simulink model "dspic_model"  (Simulink 6.4)
settings: Solver=FixedStepDiscrete  StartTime=0.0  StopTime=10.0  FixedStep=0.001  RelTol=1e-3
libraries: dsPICdrivers x8, simulink x2
CloseFcn:
  | rtwprivate ssgencode ModelCloseRequest dspic_model
settings Model: LastModifiedBy=Philipp  BufferReuse=off  ProdHWDeviceType=16-bit Generic
settings OptimizationCC: BlockReduction=off  OptimizeBlockIOStorage=off  BufferReuse=off  EnforceIntegerDowncast=off  ExpressionFolding=off  LocalBlockOutputs=off  OptimizeModelRefInitCode=on  LifeSpan=1
settings HardwareCC: ProdBitPerInt=16  ProdEndianess=LittleEndian  ProdWordSize=16  ProdHWDeviceType=16-bit Generic  TargetHWDeviceType=32-bit Generic
settings RTWCC: SystemTargetFile=dspic.tlc  TemplateMakefile=dspic_pic30_gcc.tmf  PostCodeGenCommand=dsPIC_Compile()  Description=Embedded Target for Microchip dsPIC (real-time)  ProcessScript=dspic_make_rtw_hook
settings CodeAppCC: IgnoreCustomStorageClasses=off
settings STFCustomTargetCC: TargetFcnLib=ansi_tfl_tmw.mat  GenFloatMathFcnCalls=ANSI_C  ModelReferenceCompliant=off  IncludeMdlTerminateFcn=off  CombineOutputUpdateFcns=on  SuppressErrorStatus=on  IncludeERTFirstTime=on  ERTCustomFileBanners=on  SupportContinuousTime=off  SupportNonInlinedSFcns=off  SystemTargetFile=dspic.tlc
settings ERTTargetCC: TargetFcnLib=ansi_tfl_tmw.mat  GenFloatMathFcnCalls=ANSI_C  ModelReferenceCompliant=off  IncludeMdlTerminateFcn=off  SuppressErrorStatus=on  IncludeERTFirstTime=on  ERTFirstTimeCompliant=off  InlinedParameterPlacement=NonHierarchical  ERTSrcFileBannerTemplate=dsPIC_code_template.cgt  ERTHdrFileBannerTemplate=dsPIC_code_template.cgt  ERTDataSrcFileTemplate=dsPIC_code_template.cgt  ERTDataHdrFileTemplate=dsPIC_code_template.cgt  ERTCustomFileTemplate=dsPIC_main.tlc  InitialValueSource=Model
settings CustomProperty: DataType=string  Value=C:\PROGRA~1\MATLAB\R2006a\rtw\bin\win32\gmake

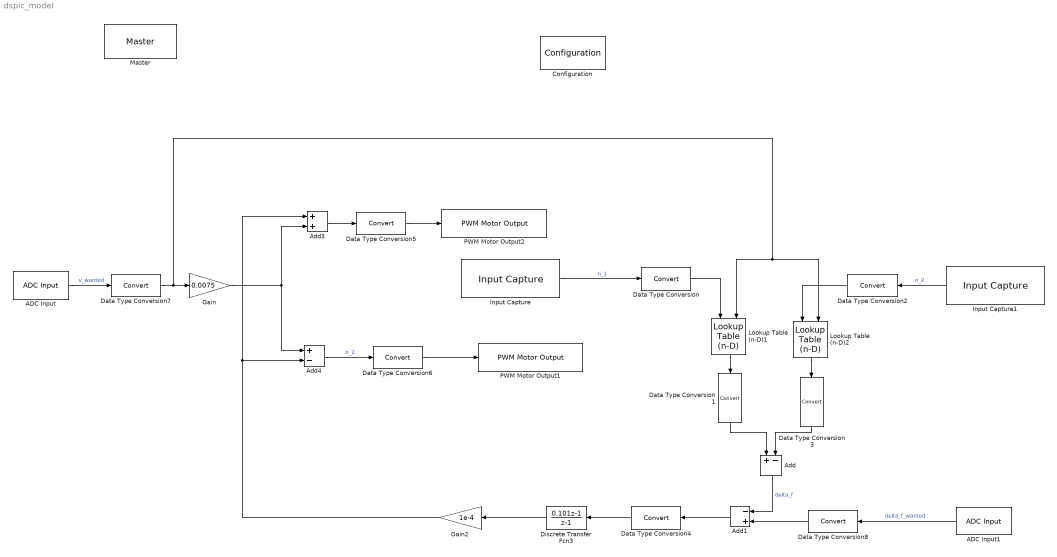
== system dspic_model ==
  ADC Input : dsPICdrivers/Peripheral I//O/ADC Input  Tag=dsPIC_ADC  Priority=5  ADC_TYPE=10 bits  ADC_MODE=Continuous sampling & get last channel value  NbrSampleStep=1  VoltRefpopup="AVdd  -  AVss"  OutFormatBitspopup=0000 00dd dddd dddd : Integer  InterruptPriority=6  ANCHANNELS=[0]  MaxName=ANmax = 1024  Rin=1e2  ADCS=0  SAMC=1  Temperature=25  SampleTime=0.001  Status="OK  |  Tsmp=5.000e-007 |  T/Channel=6.500e-006 |  Tall=6.500e-006"
  ADC Input1 : dsPICdrivers/Peripheral I//O/ADC Input  Tag=dsPIC_ADC  Orientation=left  Priority=5  ADC_TYPE=10 bits  ADC_MODE=Continuous sampling & get last channel value  NbrSampleStep=1  VoltRefpopup="AVdd  -  AVss"  OutFormatBitspopup=0000 00dd dddd dddd : Integer  InterruptPriority=6  ANCHANNELS=[1]  MaxName=ANmax = 1024  Rin=1e2  ADCS=0  SAMC=1  Temperature=25  SampleTime=0.001  Status="OK  |  Tsmp=5.000e-007 |  T/Channel=6.500e-006 |  Tall=6.500e-006"
  Add : Sum  Orientation=down  Inputs=+-  OutScaling=2^-10  SampleTime=0.001
  Add1 : Sum  Orientation=left  Inputs=-+  OutScaling=2^-10  SampleTime=0.001
  Add3 : Sum  OutScaling=2^-10  SampleTime=0.001
  Add4 : Sum  Inputs=+-  OutScaling=2^-10  SampleTime=0.001
  Configuration : dsPICdrivers/Configuration  SystemSampleTime=-1  double64=off
  Data Type Conversion : DataTypeConversion  OutDataTypeMode=double
  Data Type Conversion1 : DataTypeConversion  Orientation=down  OutDataTypeMode=uint16
  Data Type Conversion2 : DataTypeConversion  Orientation=left  OutDataTypeMode=double
  Data Type Conversion3 : DataTypeConversion  Orientation=down  OutDataTypeMode=uint16
  Data Type Conversion4 : DataTypeConversion  Orientation=left  OutDataTypeMode=double  SampleTime=0.001
  Data Type Conversion5 : DataTypeConversion  OutDataTypeMode=uint16  SampleTime=0.001
  Data Type Conversion6 : DataTypeConversion  OutDataTypeMode=uint16  SampleTime=0.001
  Data Type Conversion7 : DataTypeConversion  OutDataTypeMode=double  SampleTime=0.001
  Data Type Conversion8 : DataTypeConversion  Orientation=left  OutDataTypeMode=uint16  SampleTime=0.001
  Discrete Transfer Fcn3 : DiscreteTransferFcn  Orientation=left  Numerator=[0.101 -1]  Denominator=[1 -1]  SampleTime=0.001
  Gain : Gain  Gain=0.0075  SampleTime=0.001
  Gain2 : Gain  Orientation=left  Gain=1e-4  SampleTime=0.001
  Input Capture : dsPICdrivers/Peripheral I//O/Input Capture  Tag=dsPIC_PWM_IC  Priority=5  IntPriority=7  Channel=[ 1 ]  Channel_UP_Down_Periode=[4]  MaxChannel=[0.05]  SafeMarge=[10]  MaxName=' IC1max '  Precision=[15.6096]  Timer=[2]  ChangeDetected=[0]  ChangeDetectedPortRef=3  SampleTime=0.001  Status=OK
  Input Capture1 : dsPICdrivers/Peripheral I//O/Input Capture  Tag=dsPIC_PWM_IC  Orientation=left  Priority=5  IntPriority=7  Channel=[ 2 ]  Channel_UP_Down_Periode=[4]  MaxChannel=[0.05]  SafeMarge=[10]  MaxName=' IC2max '  Precision=[15.6096]  Timer=[2]  ChangeDetected=[0]  ChangeDetectedPortRef=3  SampleTime=0.001  Status=OK
  Lookup Table (n-D)1 : simulink/Lookup Tables/Lookup Table (n-D)  Orientation=down  numDimsPopupSelect=2  bp1=[3000 3500 4000 4500 5000 5500 6000 6500 7000 7500 8000 8500 9000 9500 10000 10500 11000 11500 12000]  bp2=[0 30]  bp3=[1:3]  bp4=[1:3]  bpcell={ [1:3], [1:3] }  explicitNumDims=2  searchMode=Binary Search  cacheBpFlag=off  vectorInputFlag=off  tableData=[1.73 -3;1.91 -3;2.55 -2.5;3.14 -2;3.6 -1.66;4.06 -1.21;4.6 -0.32;5.68 0.68;6.4 1.68;7.45 2.45;8.68 3.4;9.66 5.29;10.97 6.37;11.74 6.85;13.41 7.71;14.77 8.82;16.41 10.08;17.85 11.58;19.54 13.19]  interpMethod=Linear  extrapMethod=Linear  rangeErrorMode=None
  Lookup Table (n-D)2 : simulink/Lookup Tables/Lookup Table (n-D)  Orientation=down  numDimsPopupSelect=2  bp1=[3000 3500 4000 4500 5000 5500 6000 6500 7000 7500 8000 8500 9000 9500 10000 10500 11000 11500 12000]  bp2=[0 30]  bp3=[1:3]  bp4=[1:3]  bpcell={ [1:3], [1:3] }  explicitNumDims=2  searchMode=Binary Search  cacheBpFlag=off  vectorInputFlag=off  tableData=[1.73 -3;1.91 -3;2.55 -2.5;3.14 -2;3.6 -1.66;4.06 -1.21;4.6 -0.32;5.68 0.68;6.4 1.68;7.45 2.45;8.68 3.4;9.66 5.29;10.97 6.37;11.74 6.85;13.41 7.71;14.77 8.82;16.41 10.08;17.85 11.58;19.54 13.19]  interpMethod=Linear  extrapMethod=Linear  rangeErrorMode=None
  Master : dsPICdrivers/Master  Tag=dsPIC_MASTER  Priority=1  TimeStepType=Timer1  picType=30f3011  fcy=1e6  Quartz_33f=5e6  PLLActive_33f=off  fcyDesired_33f=0  tmr1="[1  1000  0]"  tmr1Info="Time Step : 0.001  ;   Error : 0%  PR1=1000"  tmr2345="[1  0  0  0]"  tmr2345cfg=[-1 -1 -1 -1]  IOautoConf=on  typePort="[ 0  0  0  0  0  0  0  0  0  0  0  0  0  0  0  0  8  8  0  0  0  0  0  0  0  0  0  0  0  0  0  0  0  0  0  0  0  0  0  0  0  0  0  0  0  0  0  0  6  6  0  0  0  0  0  0  0  0  0  0  0  0  0  0  0  0  0  0  0  0  0  0  0  0  0  0  0  0  0  0  0  0  0  0  0  0  0  0  0  0  0  0  0  0  0  0  0  0  0  0  0  0  0  0  0  0  0  0  0  0  0  0 ]"  TRIS="[ 65535  65535  65535  65535  65535  65535  65535 ]"  ADPCFG=0  MasterBusyPort=None  MasterOverloadPort=None  FOSC=XT  TempProtection_33f=TEMP_ON  FPBOR=PBOR_OFF  PWRT=PWRT_OFF  MCLR=MCLR_DIS  PowerSave=off
  PWM Motor Output1 : dsPICdrivers/Peripheral I//O/PWM Motor Output  Tag=dsPIC_PWM_motor  Priority=5  InputEnableChk=off  InputPeriodeChk=off  Channel=[2 ]  TPeriode=.01  PrescalerValue=1  PeriodeInteger=5000  MaxName='PWM'  Centered=on  HChannelON=off  Info="Nbr Bits : 13.2877  ||  PWM = 10000  ||  Prescaler = 1"  Delay=0  IntPriority=5  nbrPwmChannelPIC=3  Status=OK
  PWM Motor Output2 : dsPICdrivers/Peripheral I//O/PWM Motor Output  Tag=dsPIC_PWM_motor  Priority=5  InputEnableChk=off  InputPeriodeChk=off  Channel=[1]  TPeriode=.01  PrescalerValue=1  PeriodeInteger=5000  MaxName='PWM'  Centered=on  HChannelON=off  Info="Nbr Bits : 13.2877  ||  PWM = 10000  ||  Prescaler = 1"  Delay=0  IntPriority=5  nbrPwmChannelPIC=3  Status=OK
  wires:
  Discrete Transfer Fcn3/1 -> Gain2/1
  Input Capture/1 -> Data Type Conversion/1  "n_1"
  Data Type Conversion/1 -> Lookup Table (n-D)1/1
  Add/1 -> Add1/1  "delta_f"
  Input Capture1/1 -> Data Type Conversion2/1  "n_2"
  Data Type Conversion2/1 -> Lookup Table (n-D)2/1
  Data Type Conversion3/1 -> Add/2
  Data Type Conversion1/1 -> Add/1
  ADC Input1/1 -> Data Type Conversion8/1  "delta_f_wanted"
  Add1/1 -> Data Type Conversion4/1
  ADC Input/1 -> Data Type Conversion7/1  "v_wanted"
  Add4/1 -> Data Type Conversion6/1  "n_2"
  Add3/1 -> Data Type Conversion5/1
  Data Type Conversion5/1 -> PWM Motor Output2/1
  Data Type Conversion6/1 -> PWM Motor Output1/1
  Data Type Conversion4/1 -> Discrete Transfer Fcn3/1
  Data Type Conversion8/1 -> Add1/2
  Data Type Conversion7/1 -> Gain/1, Lookup Table (n-D)1/2, Lookup Table (n-D)2/2
  Gain2/1 -> Add4/2, Add3/1
  Gain/1 -> Add4/1, Add3/2
  Lookup Table (n-D)2/1 -> Data Type Conversion3/1
  Lookup Table (n-D)1/1 -> Data Type Conversion1/1
